simulink model "SAC_MPC_angle_reduced_policy"  (R2026b)
settings: Solver=ode14x  StartTime=0  StopTime=max_time  FixedStep=simStepSize
undefined symbols (not defined in the file or in its folder): driving, initialPosition, max_time, reward_Cact_d, reward_Calive, reward_Cdist, reward_Ck, reward_Crate, reward_Csteer_d, reward_Cy, reward_Cyaw, reward_Rfail, reward_Rsuccess
libraries: dspstat3 x4, drivingscenarioandsensors x2, simulink_extras x2, rllib x1
settings Model: DataDictionary=RL_data.sldd  Creator=Jacob  LastModifiedBy=scb548
settings SimscapeCC: SimscapeUseEnergyAccounting=off

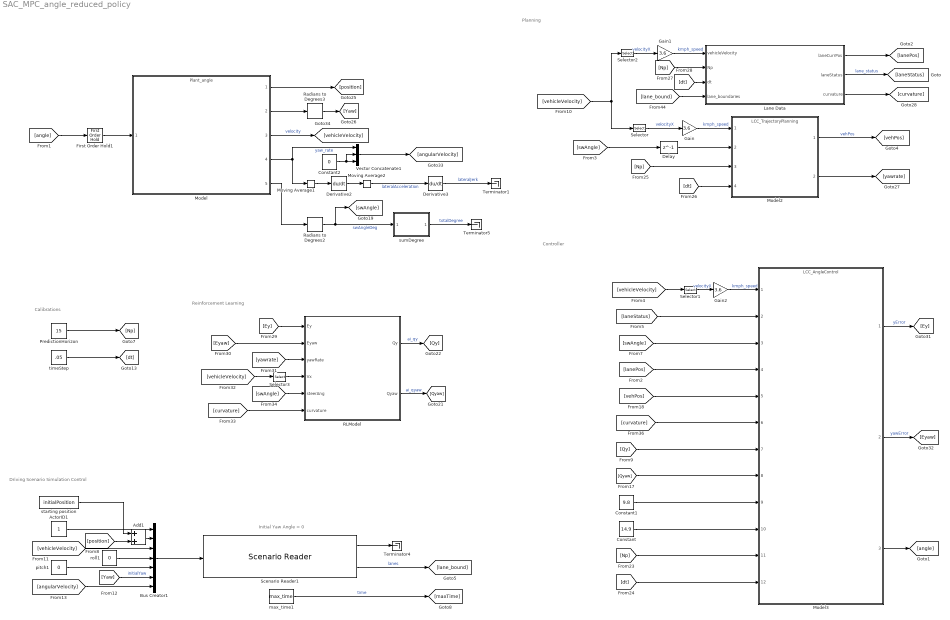
== system SAC_MPC_angle_reduced_policy ==
  note: Driving Scenario Simulation Control
  note: Reinforcement Learning
  note: Calibrations
  note: Controller
  note: Planning
  note: Initial Yaw Angle = 0
  ActorID1 : Constant
  Add1 : Sum
  Bus Creator1 : BusCreator  Inputs=7  OutDataTypeStr=Bus: BusActorPose  NonVirtualBus=on
      settings: InheritFromInputs=off
  Constant : Constant  Value=14.9
  Constant1 : Constant  Value=9.8
  Constant2 : Constant  Value=0
  Delay : Delay  DelayLength=1
  Derivative2 : Derivative
  Derivative3 : Derivative
  First Order Hold1 : FirstOrderHold  ErrorTolerance=inf  AllowContinuousInput=on
  Gain : Gain  Gain=3.6
  Gain1 : Gain  Gain=3.6
  Gain2 : Gain  Gain=3.6
  Lane Data : Subsystem
  Model : ModelReference  ModelNameDialog=Plant_angle.slx  SimulationMode=Normal  ModelReferenceVersion=7.12
  Model2 : ModelReference  ModelNameDialog=LCC_TrajectoryPlanning.slx  SimulationMode=Normal  ModelReferenceVersion=5.57
  Model3 : ModelReference  ModelNameDialog=LCC_AngleControl.slx  SimulationMode=Normal  ModelReferenceVersion=5.141
  Moving Average1 : dspstat3/Moving Average  Method=Sliding window  ForgettingFactorPort=off  SpecifyWindowLength=on  WindowLengthSource=Property  MaxWindowLength=20  WindowLength=4  OverlapLength=3  AllowArbitraryInputLength=off  ForgettingFactor=0.9  SimulateUsing=Interpreted execution
  Moving Average2 : dspstat3/Moving Average  Method=Sliding window  ForgettingFactorPort=off  SpecifyWindowLength=on  WindowLengthSource=Property  MaxWindowLength=20  WindowLength=4  OverlapLength=3  AllowArbitraryInputLength=off  ForgettingFactor=0.9  SimulateUsing=Interpreted execution
  PredictionHorizon : Constant  Value=15
  RLModel : Subsystem
  Radians to Degrees2 : simulink_extras/Transformations/Radians to Degrees
  Radians to Degrees3 : simulink_extras/Transformations/Radians to Degrees
  Scenario Reader1 : drivingscenarioandsensors/Scenario Reader  ScenarioSource=From workspace  ScenarioFileName=..\Lane Scenarios\Test_Scenario_LeftCurv.mat  ScenarioVariableName=scenario  OutputCoordinateSystem=Vehicle coordinates  EgoVehicleSource=Input port  EgoVehicleActorID=1  OrientVehiclesOnRoad=off  OutputEgoVehiclePose=off  OutputEgoVehicleState=off  SampleTime=.05  LaneBoundaryOutput=Ego vehicle lane boundaries  LaneBoundaryDistance=linspace(-150, 150, 101)  LaneBoundaryLocation=Center of lane markings  BusNameSource=Auto  BusName=BusActors  BusNumActorsSource=Scenario  BusNumActors=100  BusName2Source=Auto  BusName2=BusLaneBoundaries  BusNumLaneBoundariesSource=Scenario  BusNumLaneBoundaries=10  BusName3Source=Auto  BusName3=BusEgoActor  BusName4Source=Auto  BusName4=BusEgoState  ShowCoordinateLabels=on  SimulateUsing=Interpreted execution
  Selector{,1..3} (4 alike) : Selector  InputPortWidth=3  IndexOptions=Index vector (dialog)  Indices=1  OutputSizes=1  RuntimeRangeChecks=off
  Terminator1 : Terminator
  Terminator4 : Terminator
  Terminator5 : Terminator
  Vector Concatenate1 : Concatenate  NumInputs=3  Mode=Multidimensional array  ConcatenateDimension=2
  max_time1 : Constant  Value=max_time
  pitch1 : Constant  Value=0
  roll1 : Constant  Value=0
  starting position : Constant  Value=initialPosition
  sumDegree : MATLAB Function  TreatAsAtomicUnit=on  SystemSampleTime=.05
  timeStep : Constant  Value=.05
  wires:
  Model2/1 -> [vehPos]  "vehPos"
  [vehicleVelocity] -> Selector2/1, Selector/1
  Lane Data/2(laneStatus) -> [laneStatus]  "lane_status"
  Selector/1 -> Gain/1  "velocityX"
  Gain/1 -> Model2/1  "kmph_speed"
  Delay/1 -> Model2/2
  Lane Data/1(laneCurrPos) -> [lanePos]
  [vehicleVelocity] -> Selector1/1
  Selector1/1 -> Gain2/1  "velocityX"
  [swAngle] -> Delay/1
  [Np] -> Model2/3
  [dt] -> Model2/4
  timeStep/1 -> [dt]
  PredictionHorizon/1 -> [Np]
  [Np] -> Lane Data/2(Np)
  [dt] -> Lane Data/3(dt)
  Selector2/1 -> Gain1/1  "velocityX"
  Gain1/1 -> Lane Data/1(vehicleVelocity)  "kmph_speed"
  [Ey] -> RLModel/1(Ey)
  [Eyaw] -> RLModel/2(Eyaw)
  [yawrate] -> RLModel/3(yawRate)
  [vehicleVelocity] -> Selector3/1
  Lane Data/3(curvature) -> [curvature]
  [curvature] -> RLModel/6(curvature)
  [swAngle] -> RLModel/5(steerAng)
  Model2/2 -> [yawrate]
  Selector3/1 -> RLModel/4(Vx)
  [lane_bound] -> Lane Data/4(lane_boundaries)
  [angle] -> First Order Hold1/1
  First Order Hold1/1 -> Model/1
  Radians to Degrees2/1 -> sumDegree/1(current_angle), [swAngle]  "swAngleDeg"
  sumDegree/1(total_angle) -> Terminator5/1  "totalDegree"
  Model/4 -> Moving Average1/1, Vector Concatenate1/1  "yaw_rate"
  Vector Concatenate1/1 -> [angularVelocity]
  Radians to Degrees3/1 -> [Yaw]
  Model/3 -> [vehicleVelocity]  "velocity"
  Constant2/1 -> Vector Concatenate1/2, Vector Concatenate1/3
  Model/2 -> Radians to Degrees3/1
  Model/1 -> [position]
  Model/5 -> Radians to Degrees2/1
  RLModel/1(Qy) -> [Qy]  "ai_qy"
  RLModel/2(Qyaw) -> [Qyaw]  "ai_qyaw"
  Model3/3 -> [angle]
  Model3/2 -> [Eyaw]  "yawError"
  Model3/1 -> [Ey]  "yError"
  Gain2/1 -> Model3/1  "kmph_speed"
  [laneStatus] -> Model3/2
  [swAngle] -> Model3/3
  [lanePos] -> Model3/4
  [vehPos] -> Model3/5
  [curvature] -> Model3/6
  [Qy] -> Model3/7
  [Qyaw] -> Model3/8
  Constant1/1 -> Model3/9
  Constant/1 -> Model3/10
  [Np] -> Model3/11
  [dt] -> Model3/12
  Scenario Reader1/1 -> Terminator4/1
  [position] -> Add1/2
  starting position/1 -> Add1/1
  Add1/1 -> Bus Creator1/2
  pitch1/1 -> Bus Creator1/5
  [vehicleVelocity] -> Bus Creator1/3
  roll1/1 -> Bus Creator1/4
  Bus Creator1/1 -> Scenario Reader1/1
  [angularVelocity] -> Bus Creator1/7
  [Yaw] -> Bus Creator1/6  "initialYaw"
  ActorID1/1 -> Bus Creator1/1
  max_time1/1 -> [maxTime]  "time"
  Scenario Reader1/2 -> [lane_bound]  "lanes"
  Moving Average1/1 -> Derivative2/1
  Derivative2/1 -> Moving Average2/1
  Derivative3/1 -> Terminator1/1  "lateralJerk"
  Moving Average2/1 -> Derivative3/1  "lateralAcceleration"

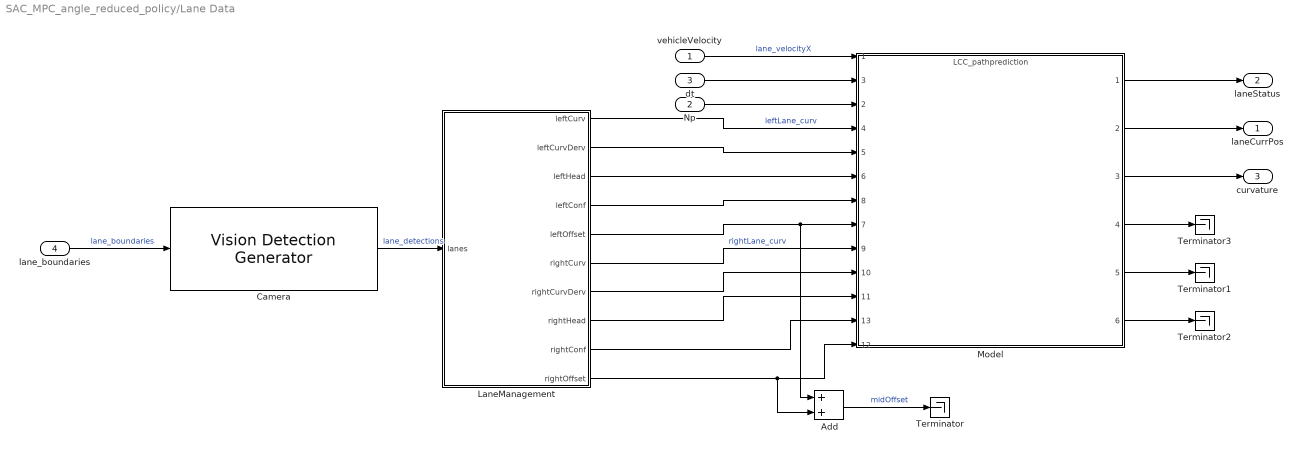
== system SAC_MPC_angle_reduced_policy/Lane Data ==
  vehicleVelocity : Inport
  Np : Inport  Port=2
  dt : Inport  Port=3
  lane_boundaries : Inport  Port=4
  Add : Sum
  Camera : drivingscenarioandsensors/Vision Detection Generator  SensorIndex=1  DetectorOutput=Lanes only  UpdateInterval=0.1  LaneUpdateInterval=0.05  SensorLocation=[1.9 0]  Height=1.1  Yaw=0  Pitch=1  Roll=0  BusNameSource=Auto  BusName=BusObjectDetections  BusName2Source=Auto  BusName2=BusLaneDetections  MaxNumDetectionsSource=Property  MaxNumDetections=50  MaxNumLanesSource=Property  MaxNumLanes=4  DetectionCoordinates=Ego Cartesian  SimulateUsing=Interpreted execution  MaxRange=150  BoundingBoxAccuracy=5  ProcessNoiseIntensity=5  MaxSpeed=100  MaxAllowedOcclusion=0.5  MinObjectImageSize=[15 15]  DetectionProbability=0.9  FalsePositivesPerImage=0.1  MinLaneImageSize=[20 3]  LaneBoundaryAccuracy=3  HasNoise=on  InitialSeedSource=Not repeatable  InitialSeed=0  UsedSeed=0  ActorProfilesSource=From Scenario Reader block  ActorProfilesParameters=driving.internal.ActorProfilesParameters  ActorProfilesExpression=[struct('ActorID',1,'ClassID',1,'Length',4.7,'Width',1.8,'Height',1.4,'OriginOffset',[-1.35 0 0],'MeshVertices',[3.7 0.9 0.857439446366782;3.7 -0.9 0.857439446366782;3.7 -0.9 0.314878892733564;3.7 0.9 0.314878892733564;3.7 0.9 0.857439446366782;2.525 0.9 0.993079584775086;2.525 -0.9 0.993079584775086;3.7 -0.9 0.857439446366782;1.82 0.72 1.4;0.41 0.72 1.4;0.41 -0.72 1.4;1.82 -0.72 1.4;-0.295 0.9 0.993079584775086;-1 0.9 0.857439446366782;-1 -0.9 0.857439446366782;-0.295 -0.9 0.993079584775086;3.7 0.9 0.857439446366782;3.7 0.9 0.314878892733564;2.525 0.9 0.314878892733564;2.525 0.9 0.993079584775086;2.525 0.9 0.993079584775086;2.525 0.9 0.314878892733564;-0.295 0.9 0.314878892733564;-0.295 0.9 0.993079584775086;-0.295 0.9 0.993079584775086;-0.295 0.9 0.314878892733564;-1 0.9 0.355570934256055;-1 0.9 0.857439446366782;2.525 0.9 0.993079584775086;-0.295 0.9 0.993079584775086;0.41 0.72 1.4;1.82 0.72 1.4;3.7 -0.9 0.857439446366782;3.7 -0.9 0.314878892733564;2.525 -0.9 0.314878892733564;2.525 -0.9 0.993079584775086;2.525 -0.9 0.993079584775086;2.525 -0.9 0.314878892733564;-0.295 -0.9 0.314878892733564;-0.295 -0.9 0.993079584775086;-0.295 -0.9 0.993079584775086;-0.295 -0.9 0.314878892733564;-1 -0.9 0.355570934256055;-1 -0.9 0.857439446366782;2.525 -0.9 0.993079584775086;-0.295 -0.9 0.993079584775086;0.41 -0.72 1.4;1.82 -0.72 1.4;-0.295 0.9 0.993079584775086;-0.295 -0.9 0.993079584775086;0.41 -0.72 1.4;0.41 0.72 1.4;2.525 -0.9 0.993079584775086;1.82 -0.72 1.4;1.82 0.72 1.4;2.525 0.9 0.993079584775086;-1 0.9 0.857439446366782;-1 0.9 0.355570934256055;-1 -0.9 0.355570934256055;-1 -0.9 0.857439446366782;3.7 0.9 0.314878892733564;3.7 -0.9 0.314878892733564;-0.295 -0.9 0.314878892733564;-0.295 0.9 0.314878892733564;-0.295 0.9 0.314878892733564;-1 0.9 0.355570934256055;-1 -0.9 0.355570934256055;-0.295 -0.9 0.314878892733564;0 -0.63 0;0 -0.87 0;0.191030206995054 -0.63 0.0601365173421445;0.191030206995054 -0.87 0.0601365173421445;0.309093367795925 -0.63 0.217575963708927;0.309093367795925 -0.87 0.217575963708927;0.309093367795925 -0.63 0.412181821758201;0.309093367795925 -0.87 0.412181821758201;0.191030206995054 -0.63 0.569621268124983;0.191030206995054 -0.87 0.569621268124983;0 -0.63 0.629757785467128;0 -0.87 0.629757785467128;-0.191030206995054 -0.63 0.569621268124983;-0.191030206995054 -0.87 0.569621268124983;-0.309093367795925 -0.63 0.412181821758201;-0.309093367795925 -0.87 0.412181821758201;-0.309093367795925 -0.63 0.217575963708927;-0.309093367795925 -0.87 0.217575963708927;-0.191030206995054 -0.63 0.0601365173421445;-0.191030206995054 -0.87 0.0601365173421445;0 -0.63 0;0 -0.87 0;0 -0.63 0;0.191030206995054 -0.63 0.0601365173421445;0.309093367795925 -0.63 0.217575963708927;0.309093367795925 -0.63 0.412181821758201;0.191030206995054 -0.63 0.569621268124983;0 -0.63 0.629757785467128;-0.191030206995054 -0.63 0.569621268124983;-0.309093367795925 -0.63 0.412181821758201;-0.309093367795925 -0.63 0.217575963708927;-0.191030206995054 -0.63 0.0601365173421445;0 -0.87 0;0.191030206995054 -0.87 0.0601365173421445;0.309093367795925 -0.87 0.217575963708927;0.309093367795925 -0.87 0.412181821758201;0.191030206995054 -0.87 0.569621268124983;0 -0.87 0.629757785467128;-0.191030206995054 -0.87 0.569621268124983;-0.309093367795925 -0.87 0.412181821758201;-0.309093367795925 -0.87 0.217575963708927;-0.191030206995054 -0.87 0.0601365173421445;0 0.87 0;0 0.63 0;0.191030206995054 0.87 0.0601365173421445;0.191030206995054 0.63 0.0601365173421445;0.309093367795925 0.87 0.217575963708927;0.309093367795925 0.63 0.217575963708927;0.309093367795925 0.87 0.412181821758201;0.309093367795925 0.63 0.412181821758201;0.191030206995054 0.87 0.569621268124983;0.191030206995054 0.63 0.569621268124983;0 0.87 0.629757785467128;0 0.63 0.629757785467128;-0.191030206995054 0.87 0.569621268124983;-0.191030206995054 0.63 0.569621268124983;-0.309093367795925 0.87 0.412181821758201;-0.309093367795925 0.63 0.412181821758201;-0.309093367795925 0.87 0.217575963708927;-0.309093367795925 0.63 0.217575963708927;-0.191030206995054 0.87 0.0601365173421445;-0.191030206995054 0.63 0.0601365173421445;0 ...(+3718 chars)],'MeshFaces',[1 2 3;3 4 1;5 6 7;7 8 5;9 10 11;11 12 9;13 14 15;15 16 13;17 18 19;19 20 17;21 22 23;23 24 21;25 26 27;27 28 25;29 30 31;31 32 29;33 34 35;35 36 33;37 38 39;39 40 37;41 42 43;43 44 41;45 46 47;47 48 45;49 50 51;51 52 49;53 54 55;55 56 53;57 58 59;59 60 57;61 62 63;63 64 61;65 66 67;67 68 65;69 71 72;72 70 69;71 73 74;74 72 71;73 75 76;76 74 73;75 77 78;78 76 75;77 79 80;80 78 77;79 81 82;82 80 79;81 83 84;84 82 81;83 85 86;86 84 83;85 87 88;88 86 85;87 89 90;90 88 87;91 92 93;91 93 94;91 94 95;91 95 96;91 96 97;91 97 98;91 98 99;91 99 100;101 102 103;101 103 104;101 104 105;101 105 106;101 106 107;101 107 108;101 108 109;101 109 110;111 113 114;114 112 111;113 115 116;116 114 113;115 117 118;118 116 115;117 119 120;120 118 117;119 121 122;122 120 119;121 123 124;124 122 121;123 125 126;126 124 123;125 127 128;128 126 125;127 129 130;130 128 127;129 131 132;132 130 129;133 134 135;133 135 136;133 136 137;133 137 138;133 138 139;133 139 140;133 140 141;133 141 142;143 144 145;143 145 146;143 146 147;143 147 148;143 148 149;143 149 150;143 150 151;143 151 152;153 155 156;156 154 153;155 157 158;158 156 155;157 159 160;160 158 157;159 161 162;162 160 159;161 163 164;164 162 161;163 165 166;166 164 163;165 167 168;168 166 165;167 169 170;170 168 167;169 171 172;172 170 169;171 173 174;174 172 171;175 176 177;175 177 178;175 178 179;175 179 180;175 180 181;175 181 182;175 182 183;175 183 184;185 186 187;185 187 188;185 188 189;185 189 190;185 190 191;185 191 192;185 192 193;185 193 194;195 197 198;198 196 195;197 199 200;200 198 197;199 201 202;202 200 199;201 203 204;204 202 201;203 205 206;206 204 203;205 207 208;208 206 205;207 209 210;210 208 207;209 211 212;212 210 209;211 213 214;214 212 211;213 215 216;216 214 213;217 218 219;217 219 220;217 220 221;217 221 222;217 222 223;217 223 224;217 224 225;217 225 226;227 228 229;227 229 230;227 230 231;227 231 232;227 232 233;227 233 234;227 234 235;227 235 236],'RCSPattern',[10 10;10 10],'RCSAzimuthAngles',[-180 180],'RCSElevationAngles',[-90 90])]  Intrinsics=driving.internal.cameraIntrinsics('FocalLength',[800 800],'PrincipalPoint',[320 240],'ImageSize',[480 640],'RadialDistortion',[0 0],'TangentialDistortion',[0 0],'Skew',0)
  LaneManagement : MATLAB Function  TreatAsAtomicUnit=on
  Model : ModelReference  ModelNameDialog=LCC_pathprediction.slx  SimulationMode=Normal  ModelReferenceVersion=5.69
      settings: PortSchema="{\"entries\":[{\"content\":{\"sides\":[{\"content\":{\"connectorIds\":[\"In1\",\"In3\",\"In2\",\"In4\",\"In5\",\"In6\",\"In8\",\"In7\",\"In9\",\"In10\",\"In11\",\"In13\",\"In12\"]},\"type\":\"ConnectorPlacement.EquallySpacedRectSide\",\"uuid\":\"a07f8485-8c73-44ce-93cf-ec5e6f63c5da\"},{\"content\":{\"connectorIds\":[\"Out1\",\"Out2\",\"Out3\",\"Out4\",\"Out5\",\"Out6\"],\"side\":\"RIGHT\"},\"type\":\"ConnectorPlacement.EquallySpacedRectSide\",\"uuid\":\"b69156b0-73a0-4176-8c64-fda440ac3685\"},{\"content\":{\"side\":\"TOP\"},\"type\":\"ConnectorPlacement.EquallySpacedRectSide\",\"uuid\":\"33404bc1-182d-48ae-8070-d21d23a4a197\"}]},\"type\":\"ConnectorPlacement.EquallySpacedConnector\",\"uuid\":\"de203df0-0780-4dcc-b040-a4939f0923fa\"}],\"packageUris\":[\"http://schema.mathworks.com/mf0/Connector/R2020b\"],\"version\":\"1.0\"}"
  Terminator{,1..3} (4 alike) : Terminator
  laneCurrPos : Outport
  laneStatus : Outport  Port=2
  curvature : Outport  Port=3
  wires:
  Model/1 -> laneStatus/1
  Model/2 -> laneCurrPos/1
  Model/3 -> curvature/1
  vehicleVelocity/1 -> Model/1  "lane_velocityX"
  Np/1 -> Model/2
  dt/1 -> Model/3
  Model/5 -> Terminator1/1
  LaneManagement/1(leftCurv) -> Model/4  "leftLane_curv"
  LaneManagement/2(leftCurvDerv) -> Model/5
  LaneManagement/3(leftHead) -> Model/6
  LaneManagement/4(leftConf) -> Model/8
  LaneManagement/5(leftOffset) -> Add/1, Model/7
  LaneManagement/6(rightCurv) -> Model/9  "rightLane_curv"
  LaneManagement/10(rightOffset) -> Model/12, Add/2
  LaneManagement/9(rightConf) -> Model/13
  LaneManagement/8(rightHead) -> Model/11
  LaneManagement/7(rightCurvDerv) -> Model/10
  Camera/1 -> LaneManagement/1(lanes)  "lane_detections"
  lane_boundaries/1 -> Camera/1  "lane_boundaries"
  Model/6 -> Terminator2/1
  Model/4 -> Terminator3/1
  Add/1 -> Terminator/1  "midOffset"

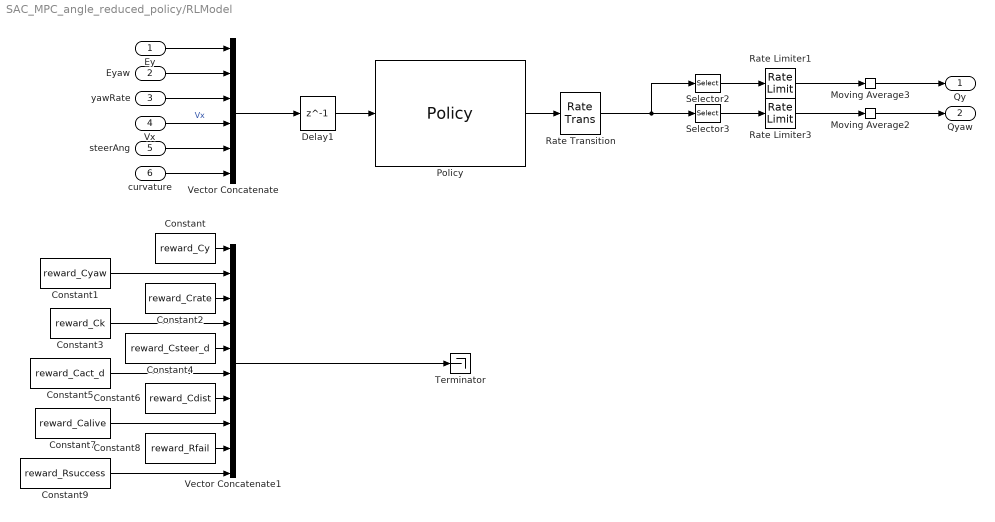
== system SAC_MPC_angle_reduced_policy/RLModel ==
  Ey : Inport
  Eyaw : Inport  Port=2
  yawRate : Inport  Port=3
  Vx : Inport  Port=4
  steerAng : Inport  Port=5
  curvature : Inport  Port=6
  Constant : Constant  Value=reward_Cy
  Constant1 : Constant  Value=reward_Cyaw
  Constant2 : Constant  Value=reward_Crate
  Constant3 : Constant  Value=reward_Ck
  Constant4 : Constant  Value=reward_Csteer_d
  Constant5 : Constant  Value=reward_Cact_d
  Constant6 : Constant  Value=reward_Cdist
  Constant7 : Constant  Value=reward_Calive
  Constant8 : Constant  Value=reward_Rfail
  Constant9 : Constant  Value=reward_Rsuccess
  Delay1 : Delay  DelayLength=1
  Moving Average2 : dspstat3/Moving Average  Method=Sliding window  ForgettingFactorPort=off  SpecifyWindowLength=on  WindowLengthSource=Property  MaxWindowLength=20  WindowLength=5  OverlapLength=4  AllowArbitraryInputLength=off  ForgettingFactor=0.9  SimulateUsing=Interpreted execution
  Moving Average3 : dspstat3/Moving Average  Method=Sliding window  ForgettingFactorPort=off  SpecifyWindowLength=on  WindowLengthSource=Property  MaxWindowLength=20  WindowLength=5  OverlapLength=4  AllowArbitraryInputLength=off  ForgettingFactor=0.9  SimulateUsing=Interpreted execution
  Policy : rllib/Policy  MATFile=reducedAgent_policy.mat  PolicyParamsAsInput=off  PolicyParamsBusName=policy_param_bus  SimUsingCodegen=off
  Rate Limiter1 : RateLimiter  RisingSlewLimit=.5  FallingSlewLimit=-.5  SampleTimeMode=inherited
  Rate Limiter3 : RateLimiter  RisingSlewLimit=.5  FallingSlewLimit=-.5  SampleTimeMode=inherited
  Rate Transition : RateTransition  InitialCondition=.1  OutPortSampleTime=.05
  Selector2 : Selector  InputPortWidth=2  IndexOptions=Index vector (dialog)  Indices=1  OutputSizes=1  RuntimeRangeChecks=off
  Selector3 : Selector  InputPortWidth=2  IndexOptions=Index vector (dialog)  Indices=2  OutputSizes=1  RuntimeRangeChecks=off
  Terminator : Terminator
  Vector Concatenate : Concatenate  NumInputs=6  Mode=Multidimensional array
  Vector Concatenate1 : Concatenate  NumInputs=10
  Qy : Outport
  Qyaw : Outport  Port=2
  wires:
  Vector Concatenate/1 -> Delay1/1
  steerAng/1 -> Vector Concatenate/5
  Policy/1 -> Rate Transition/1
  curvature/1 -> Vector Concatenate/6
  yawRate/1 -> Vector Concatenate/3
  Vx/1 -> Vector Concatenate/4  "Vx"
  Ey/1 -> Vector Concatenate/1
  Eyaw/1 -> Vector Concatenate/2
  Selector3/1 -> Rate Limiter3/1
  Selector2/1 -> Rate Limiter1/1
  Rate Transition/1 -> Selector2/1, Selector3/1
  Delay1/1 -> Policy/1
  Rate Limiter3/1 -> Moving Average2/1
  Rate Limiter1/1 -> Moving Average3/1
  Moving Average2/1 -> Qyaw/1
  Moving Average3/1 -> Qy/1
  Constant4/1 -> Vector Concatenate1/5
  Constant5/1 -> Vector Concatenate1/6
  Constant3/1 -> Vector Concatenate1/4
  Constant9/1 -> Vector Concatenate1/10
  Constant2/1 -> Vector Concatenate1/3
  Constant6/1 -> Vector Concatenate1/7
  Constant7/1 -> Vector Concatenate1/8
  Constant1/1 -> Vector Concatenate1/2
  Vector Concatenate1/1 -> Terminator/1
  Constant/1 -> Vector Concatenate1/1
  Constant8/1 -> Vector Concatenate1/9

== matlab function SAC_MPC_angle_reduced_policy/sumDegree ==
  data: current_angle input; total_angle output
function total_angle = angle_calc(current_angle)

% add change in angle to the total angle
persistent angle
persistent angle_old

if isempty(angle)
    angle = 0;
end
if isempty(angle_old)
    angle_old = 0;
end

difference  = abs(angle_old - current_angle);

angle = angle + difference;

total_angle = angle;

angle_old = current_angle;

== matlab function SAC_MPC_angle_reduced_policy/Lane Data/LaneManagement ==
  data: lanes input size=[1 1]; leftCurv output; leftCurvDerv output; leftHead output; leftConf output; leftOffset output; rightCurv output; rightCurvDerv output; rightHead output; rightConf output; rightOffset output
function [leftCurv, leftCurvDerv, leftHead, leftConf, leftOffset, rightCurv, rightCurvDerv, rightHead, rightConf, rightOffset] = LaneManagement(lanes)

leftCurv = 0;
leftCurvDerv = 0;
leftHead = 0;
leftConf = 0;
leftOffset = 0;

rightCurv = 0;
rightCurvDerv = 0;
rightHead = 0;
rightConf = 0;
rightOffset = 0;

for i=1:lanes.NumLaneBoundaries
    
    if (lanes.LaneBoundaries(i).LateralOffset > 0) && (lanes.LaneBoundaries(i).LateralOffset < 5)
        leftCurv = double(lanes.LaneBoundaries(i).Curvature);
        leftCurvDerv = double(lanes.LaneBoundaries(i).CurvatureDerivative);
        leftHead = double(lanes.LaneBoundaries(i).HeadingAngle);
        leftOffset = double(lanes.LaneBoundaries(i).LateralOffset);
        leftConf = double(1);

    elseif (lanes.LaneBoundaries(i).LateralOffset < 0) && (lanes.LaneBoundaries(i).LateralOffset > -5)
        rightCurv = double(lanes.LaneBoundaries(i).Curvature);
        rightCurvDerv = double(lanes.LaneBoundaries(i).CurvatureDerivative);
        rightHead = double(lanes.LaneBoundaries(i).HeadingAngle);
        rightOffset = double(lanes.LaneBoundaries(i).LateralOffset);
        rightConf = double(1);
    end


end
